simulink model "Modelo_Lazo_Cerrado"  (R2026b)
settings: Solver=VariableStepAuto
values from neighbouring files (symbols this model uses):
  g = 9.80665    [coeficientes.m]
settings Model: Creator=fedeb  LastModifiedBy=fedeb

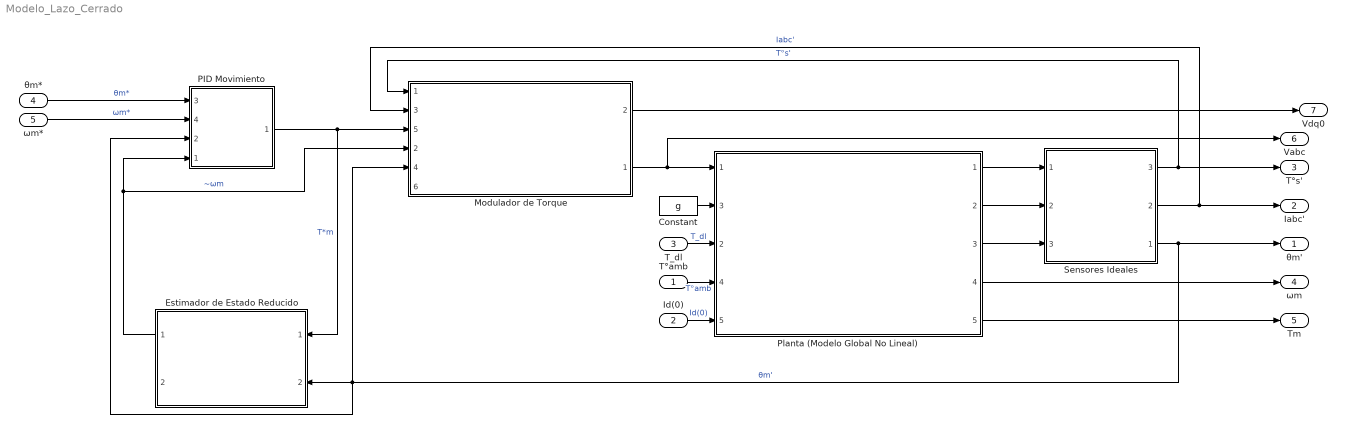
== system Modelo_Lazo_Cerrado ==
  T°amb : Inport
  Id(0) : Inport  Port=2
  T_dl : Inport  Port=3
  θm* : Inport  Port=4
  ωm* : Inport  Port=5
  Constant : Constant  Value=g
  Estimador de Estado Reducido : Subsystem  ReferencedSubsystem=Estimador_Estado_Reducido
  Modulador de Torque : Subsystem  ReferencedSubsystem=Modulador_Torque_Equivalente
      settings: PortSchema="{\"entries\":[{\"content\":{\"sides\":[{\"content\":{\"connectorIds\":[\"In1\",\"In3\",\"In5\",\"In2\",\"In4\",\"In6\"]},\"type\":\"ConnectorPlacement.EquallySpacedRectSide\",\"uuid\":\"ea9ad4ab-f607-4d37-9442-85f6cfda2486\"},{\"content\":{\"connectorIds\":[\"Out2\",\"Out1\"],\"side\":\"RIGHT\"},\"type\":\"ConnectorPlacement.EquallySpacedRectSide\",\"uuid\":\"696b5fe5-1f6c-4fc9-932e-86b56d49996f\"},{\"content\":{\"side\":\"TOP\"},\"type\":\"ConnectorPlacement.EquallySpacedRectSide\",\"uuid\":\"45e3ac4c-5a2f-4a79-9454-e497b07295c7\"}]},\"type\":\"ConnectorPlacement.EquallySpacedConnector\",\"uuid\":\"ad401c21-3c60-4ab4-96eb-f449fc93609a\"}],\"packageUris\":[\"http://schema.mathworks.com/mf0/Connector/R2020b\"],\"version\":\"1.0\"}"
  PID Movimiento : Subsystem  ReferencedSubsystem=PID_Mov
      settings: PortSchema="{\"entries\":[{\"content\":{\"sides\":[{\"content\":{\"connectorIds\":[\"In3\",\"In4\",\"In2\",\"In1\"]},\"type\":\"ConnectorPlacement.EquallySpacedRectSide\",\"uuid\":\"99b9ec4b-f651-40ed-8a16-085c2c4ac88d\"},{\"content\":{\"connectorIds\":[\"Out1\"],\"side\":\"RIGHT\"},\"type\":\"ConnectorPlacement.EquallySpacedRectSide\",\"uuid\":\"009a9369-fd86-4ac2-a423-7c7f1491457b\"},{\"content\":{\"side\":\"TOP\"},\"type\":\"ConnectorPlacement.EquallySpacedRectSide\",\"uuid\":\"0bc889a5-9100-482e-a11a-4c36993d76f7\"}]},\"type\":\"ConnectorPlacement.EquallySpacedConnector\",\"uuid\":\"de270b8a-8a15-46e7-87f3-10db7988a399\"}],\"packageUris\":[\"http://schema.mathworks.com/mf0/Connector/R2020b\"],\"version\":\"1.0\"}"
  Planta (Modelo Global No Lineal) : Subsystem  ReferencedSubsystem=Modelo_Global_NL
      settings: PortSchema="{\"entries\":[{\"content\":{\"sides\":[{\"content\":{\"connectorIds\":[\"In1\",\"In3\",\"In2\",\"In4\",\"In5\"]},\"type\":\"ConnectorPlacement.EquallySpacedRectSide\",\"uuid\":\"3481abf0-b0cb-49f6-b93f-5a31fbfa4119\"},{\"content\":{\"connectorIds\":[\"Out1\",\"Out2\",\"Out3\",\"Out4\",\"Out5\"],\"side\":\"RIGHT\"},\"type\":\"ConnectorPlacement.EquallySpacedRectSide\",\"uuid\":\"81dbc61e-d5f3-4edc-bc73-ec3d6160a008\"},{\"content\":{\"side\":\"TOP\"},\"type\":\"ConnectorPlacement.EquallySpacedRectSide\",\"uuid\":\"48e37594-92fb-4835-b4aa-9211b8b6a309\"}]},\"type\":\"ConnectorPlacement.EquallySpacedConnector\",\"uuid\":\"6c32b8e1-5803-41f4-af4e-ba3a494349ba\"}],\"packageUris\":[\"http://schema.mathworks.com/mf0/Connector/R2020b\"],\"version\":\"1.0\"}"
  Sensores Ideales : Subsystem  ReferencedSubsystem=Sensores_Ideales
      settings: PortSchema="{\"entries\":[{\"content\":{\"sides\":[{\"content\":{\"connectorIds\":[\"In1\",\"In2\",\"In3\"]},\"type\":\"ConnectorPlacement.EquallySpacedRectSide\",\"uuid\":\"f4bb6189-c8cb-4d3e-a45f-895d59b6a7f9\"},{\"content\":{\"connectorIds\":[\"Out3\",\"Out2\",\"Out1\"],\"side\":\"RIGHT\"},\"type\":\"ConnectorPlacement.EquallySpacedRectSide\",\"uuid\":\"4fe23da4-d7b3-4116-8a5c-3a889a14c1ed\"},{\"content\":{\"side\":\"TOP\"},\"type\":\"ConnectorPlacement.EquallySpacedRectSide\",\"uuid\":\"3a675bb7-2a54-45fb-91cd-5f3dc1d0d742\"}]},\"type\":\"ConnectorPlacement.EquallySpacedConnector\",\"uuid\":\"fa703284-8060-4ab8-a349-fe5cb05f502a\"}],\"packageUris\":[\"http://schema.mathworks.com/mf0/Connector/R2020b\"],\"version\":\"1.0\"}"
  θm' : Outport
  Iabc' : Outport  Port=2  OutDataTypeStr=Bus: Iabc
  T°s' : Outport  Port=3
  ωm : Outport  Port=4
  Tm : Outport  Port=5
  Vabc : Outport  Port=6  OutDataTypeStr=Bus: Vabc
  Vdq0 : Outport  Port=7  OutDataTypeStr=Bus: Vdq0
  wires:
  Planta (Modelo Global No Lineal)/1 -> Sensores Ideales/1
  Sensores Ideales/1 -> Modulador de Torque/4, PID Movimiento/2, Estimador de Estado Reducido/2, θm'/1  "θm'"
  PID Movimiento/1 -> Estimador de Estado Reducido/1, Modulador de Torque/5  "T*m"
  Planta (Modelo Global No Lineal)/2 -> Sensores Ideales/2
  Modulador de Torque/1 -> Vabc/1, Planta (Modelo Global No Lineal)/1
  Estimador de Estado Reducido/1 -> PID Movimiento/1, Modulador de Torque/2  "~ωm"
  Planta (Modelo Global No Lineal)/3 -> Sensores Ideales/3
  Sensores Ideales/2 -> Iabc'/1, Modulador de Torque/3  "Iabc'"
  Sensores Ideales/3 -> Modulador de Torque/1, T°s'/1  "T°s'"
  Constant/1 -> Planta (Modelo Global No Lineal)/3
  Id(0)/1 -> Planta (Modelo Global No Lineal)/5  "Id(0)"
  T°amb/1 -> Planta (Modelo Global No Lineal)/4  "T°amb"
  T_dl/1 -> Planta (Modelo Global No Lineal)/2  "T_dl"
  Planta (Modelo Global No Lineal)/5 -> Tm/1
  Planta (Modelo Global No Lineal)/4 -> ωm/1
  Modulador de Torque/2 -> Vdq0/1
  θm*/1 -> PID Movimiento/3  "θm*"
  ωm*/1 -> PID Movimiento/4  "ωm*"
